simulink model "HFMA_4B_1_5_9_13"  (R2026b)
settings: Solver=FixedStepDiscrete  StopTime=stopTime  FixedStep=Ts
PreLoadFcn:
  | load('a_luts.mat')
values from neighbouring files (symbols this model uses):
  cosLUT = [1 1 1 1 1 1 1 1 1 1 1 1 ... (640 elements, 16x40)]    [iq_luts.mat]
  k_avg = 10    [Simulink_DOA_Test.m]    (also in collect_ranges.m; optimised_error_code.m)
  sinLUT = [0 0 0 0 0 0 0 0 0 0 0 0 ... (640 elements, 16x40)]    [iq_luts.mat]
  Ts = 1/8000    (= 0.000125)    [Simulink_DOA_Test.m]    (also in collect_ranges.m; optimised_error_code.m)
undefined symbols (not defined in the file or in its folder): a2_Im, a2_Re, a3_Im, a3_Re, NumBits1, NumBits2, Slope1, Slope2
libraries: hdlsllib x4, sl_signal_attributes x2
(part 1 of 6)
settings Model: FPTRunName=BaselineRun  FPTShortcutValueString='{{},{''BaselineRun_2'',1,1,1,''BaselineRun_2'','''',{},''M'',''D'',''''}}'  MinMaxOverflowArchiveMode=Merge  Creator=Kayla  LastModifiedBy=Kayla
settings OptimizationCC: BlockReduction=off  ConditionallyExecuteInputs=off  DefaultParameterBehavior=Inlined  InheritOutputTypeSmallerThanSingle=on
settings DebuggingCC: ArtificialAlgebraicLoopMsg=error  IntegerOverflowMsg=none  IntegerSaturationMsg=none  ParameterPrecisionLossMsg=none  SignalRangeChecking=warning  SingleTaskRateTransMsg=error
settings HardwareCC: ProdEndianess=Unspecified  ProdEqTarget=off  ProdHWDeviceType=ASIC/FPGA->ASIC/FPGA  ProdIntDivRoundTo=Undefined  ProdLargestAtomicFloat=None  TargetEndianess=LittleEndian  TargetHWDeviceType=Custom Processor->MATLAB Host Computer  TargetIntDivRoundTo=Zero  TargetLongLongMode=on

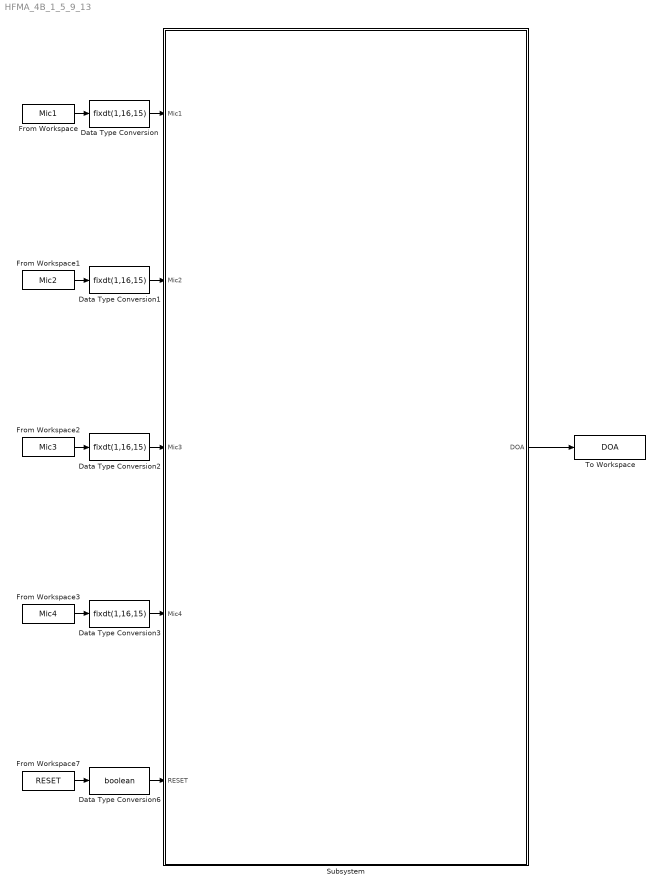
== system HFMA_4B_1_5_9_13 ==
  Data Type Conversion{,1..3} (4 alike) : DataTypeConversion  OutDataTypeStr=fixdt(1,16,15)  RndMeth=Nearest
  Data Type Conversion6 : DataTypeConversion  OutDataTypeStr=boolean  RndMeth=Nearest
  From Workspace : FromWorkspace  VariableName=Mic1  SampleTime=Ts  Interpolate=off  OutputAfterFinalValue=Holding final value
  From Workspace1 : FromWorkspace  VariableName=Mic2  SampleTime=Ts  Interpolate=off  OutputAfterFinalValue=Holding final value
  From Workspace2 : FromWorkspace  VariableName=Mic3  SampleTime=Ts  Interpolate=off  OutputAfterFinalValue=Holding final value
  From Workspace3 : FromWorkspace  VariableName=Mic4  SampleTime=Ts  Interpolate=off  OutputAfterFinalValue=Holding final value
  From Workspace7 : FromWorkspace  VariableName=RESET  SampleTime=Ts
  Subsystem : Subsystem
  To Workspace : ToWorkspace  VariableName=DOA  SaveFormat=Timeseries  SampleTime=-1
  wires:
  From Workspace7/1 -> Data Type Conversion6/1
  Subsystem/1(DOA) -> To Workspace/1
  From Workspace/1 -> Data Type Conversion/1
  From Workspace1/1 -> Data Type Conversion1/1
  From Workspace2/1 -> Data Type Conversion2/1
  From Workspace3/1 -> Data Type Conversion3/1
  Data Type Conversion/1 -> Subsystem/1(Mic1)
  Data Type Conversion1/1 -> Subsystem/2(Mic2)
  Data Type Conversion2/1 -> Subsystem/3(Mic3)
  Data Type Conversion3/1 -> Subsystem/4(Mic4)
  Data Type Conversion6/1 -> Subsystem/5(RESET)

== system HFMA_4B_1_5_9_13/Subsystem ==
  Mic1 : Inport  OutDataTypeStr=fixdt(1,16,15)  SampleTime=Ts
  Mic2 : Inport  Port=2  OutDataTypeStr=fixdt(1,16,15)  SampleTime=Ts
  Mic3 : Inport  Port=3  OutDataTypeStr=fixdt(1,16,15)  SampleTime=Ts
  Mic4 : Inport  Port=4  OutDataTypeStr=fixdt(1,16,15)  SampleTime=Ts
  RESET : Inport  Port=5  SampleTime=Ts
  A Counter : Subsystem  mask(Counter Limited){uplimit=180, tsamp=Ts}
      mask prompts: uplimit "Simulink:masks:UpperLimit_MP"; tsamp "Simulink:masks:SampleTime_MP"
      mask help: Simulink:masks:CounterLimited_MD
      mask init:
      | nbits = sl('counter_init', uplimit, gcbh);
  Add : Sum  Inputs=++++  OutDataTypeStr=fixdt(0,40,34)  SaturateOnIntegerOverflow=on
  Bandpass Filter : Subsystem
  Bandpass Filter1 : Subsystem
  Bandpass Filter2 : Subsystem
  Bandpass Filter3 : Subsystem
  Constant1 : Constant  OutDataTypeStr=fixdt(0,18,0)
  Constant13 : Constant  Value=13  OutDataTypeStr=fixdt(0,18,0)
  Constant5 : Constant  Value=5  OutDataTypeStr=fixdt(0,18,0)
  Constant9 : Constant  Value=9  OutDataTypeStr=fixdt(0,18,0)
  HFMA1 : Subsystem
  HFMA13 : Subsystem
  HFMA5 : Subsystem
  HFMA9 : Subsystem
  IQ Counter : Subsystem  mask(Counter Limited){uplimit=39, tsamp=Ts}
      mask prompts: uplimit "Simulink:masks:UpperLimit_MP"; tsamp "Simulink:masks:SampleTime_MP"
      mask help: Simulink:masks:CounterLimited_MD
      mask init:
      | nbits = sl('counter_init', uplimit, gcbh);
  Max Theta Selector : Subsystem
      settings: PortSchema="{\"entries\":[{\"content\":{\"sides\":[{\"content\":{\"connectorIds\":[\"In1\",\"In2\"]},\"type\":\"ConnectorPlacement.EquallySpacedRectSide\",\"uuid\":\"52f73d59-b961-46ba-95ec-da8ce9ae0879\"},{\"content\":{\"connectorIds\":[\"Out1\"],\"side\":\"RIGHT\"},\"type\":\"ConnectorPlacement.EquallySpacedRectSide\",\"uuid\":\"e217b0cb-9215-4a6d-97a8-b302314659a3\"},{\"content\":{\"connectorIds\":[\"In3\"],\"side\":\"TOP\"},\"type\":\"ConnectorPlacement.EquallySpacedRectSide\",\"uuid\":\"d49e545c-3ad9-445b-9897-a9fe5aaea0e6\"}]},\"type\":\"ConnectorPlacement.EquallySpacedConnector\",\"uuid\":\"e5954731-cd34-4517-a2ca-3982d6e46876\"}],\"packageUris\":[\"http://schema.mathworks.com/mf0/Connector/R2020b\"],\"version\":\"1.0\"}"
  DOA : Outport
  wires:
  Mic4/1 -> Bandpass Filter3/1(In1)
  Mic2/1 -> Bandpass Filter1/1(In1)
  Mic3/1 -> Bandpass Filter2/1(In1)
  Add/1 -> Max Theta Selector/1(P_Theta)
  Mic1/1 -> Bandpass Filter/1(Raw Signal In)
  Max Theta Selector/1(Strongest Angle) -> DOA/1
  Constant1/1 -> HFMA1/6(F0 Index)
  Constant5/1 -> HFMA5/6(F0 Index)
  Bandpass Filter/1(Filtered Output) -> HFMA1/1(Mic1), HFMA5/1(Mic1), HFMA9/1(Mic1), HFMA13/1(Mic1)
  Bandpass Filter1/1(Microphone Input) -> HFMA1/2(Mic2), HFMA5/2(Mic2), HFMA9/2(Mic2), HFMA13/2(Mic2)
  Bandpass Filter2/1(Microphone Input) -> HFMA1/3(Mic3), HFMA5/3(Mic3), HFMA9/3(Mic3), HFMA13/3(Mic3)
  Constant13/1 -> HFMA13/6(F0 Index)
  IQ Counter/1(y) -> HFMA1/7(IQ Counter), HFMA5/7(IQ Counter), HFMA9/7(IQ Counter), HFMA13/7(IQ Counter)
  A Counter/1(y) -> HFMA1/8(A Counter), HFMA5/8(A Counter), HFMA9/8(A Counter), HFMA13/8(A Counter)
  Constant9/1 -> HFMA9/6(F0 Index)
  Bandpass Filter3/1(Microphone Input) -> HFMA1/4(Mic4), HFMA5/4(Mic4), HFMA9/4(Mic4), HFMA13/4(Mic4)
  HFMA5/2(Theta) -> Max Theta Selector/2(Theta)
  RESET/1 -> Max Theta Selector/3(RESET), HFMA1/5(RESET), HFMA5/5(RESET), HFMA9/5(RESET), HFMA13/5(RESET)
  HFMA1/1(P_theta) -> Add/1
  HFMA5/1(P_theta) -> Add/2
  HFMA9/1(P_theta) -> Add/3
  HFMA13/1(P_theta) -> Add/4

== system HFMA_4B_1_5_9_13/Subsystem/A Counter ==
  Data Type Propagation : sl_signal_attributes/Data Type Propagation  PropDataTypeMode=Specify via dialog  PropDataType=uint(nbits)  IfRefDouble=double  IfRefSingle=single  IsSigned=IsSigned1 or IsSigned2  NumBitsBase=max([NumBits1 NumBits2])  NumBitsMult=1  NumBitsAdd=0  NumBitsAllowFinal=-1  PropScalingMode=Specify via dialog  PropScaling=1  ValuesUsedBestPrec=[5 -7]  SlopeBase=min([Slope1 Slope2])  SlopeMult=1  SlopeAdd=0  BiasBase=Bias1  BiasMult=1  BiasAdd=0
  Force to be scalar : SignalSpecification  DisableCoverage=on  Dimensions=1
  Increment Real World : hdlsllib/Math Operations/Increment Real World
  Output : UnitDelay  InitialCondition=0.0  SampleTime=tsamp
  Wrap To Zero : hdlsllib/Discontinuities/Wrap To Zero  Threshold=uplimit
  y : Outport
  wires:
  Increment Real World/1 -> Wrap To Zero/1
  Force to be scalar/1 -> Increment Real World/1
  Output/1 -> Force to be scalar/1, y/1
  Wrap To Zero/1 -> Output/1, Data Type Propagation/3, Data Type Propagation/2, Data Type Propagation/1

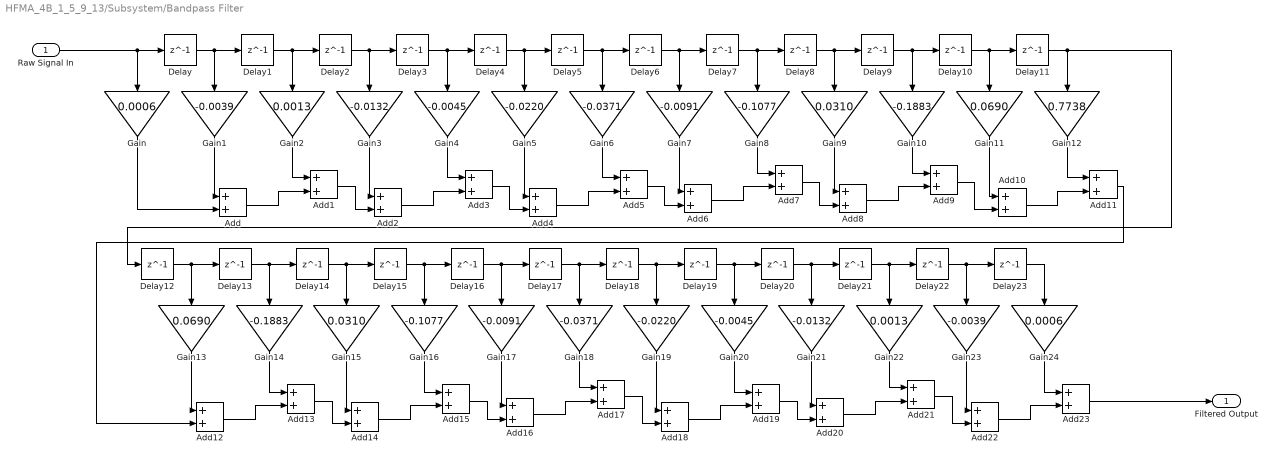
== system HFMA_4B_1_5_9_13/Subsystem/Bandpass Filter ==
  Raw Signal In : Inport
  Add{,1..23} (24 alike) : Sum  OutDataTypeStr=fixdt(1,20,17)  SaturateOnIntegerOverflow=on
  Delay{,1..23} (24 alike) : Delay  DelayLength=1
  Gain : Gain  Gain=0.0006  ParamDataTypeStr=fixdt(0,18,28)  OutDataTypeStr=fixdt(1,18,27)  SaturateOnIntegerOverflow=on
  Gain1 : Gain  Gain=-0.0039  ParamDataTypeStr=fixdt(1,18,25)  OutDataTypeStr=fixdt(1,18,24)  SaturateOnIntegerOverflow=on
  Gain10 : Gain  Gain=-0.1883  ParamDataTypeStr=fixdt(1,18,19)  OutDataTypeStr=fixdt(1,18,19)  SaturateOnIntegerOverflow=on
  Gain11 : Gain  Gain=0.0690  ParamDataTypeStr=fixdt(0,18,21)  OutDataTypeStr=fixdt(1,18,20)  SaturateOnIntegerOverflow=on
  Gain12 : Gain  Gain=0.7738  ParamDataTypeStr=fixdt(0,18,18)  OutDataTypeStr=fixdt(1,18,17)  SaturateOnIntegerOverflow=on
  Gain13 : Gain  Gain=0.0690  ParamDataTypeStr=fixdt(0,18,21)  OutDataTypeStr=fixdt(1,18,20)  SaturateOnIntegerOverflow=on
  Gain14 : Gain  Gain=-0.1883  ParamDataTypeStr=fixdt(1,18,19)  OutDataTypeStr=fixdt(1,18,19)  SaturateOnIntegerOverflow=on
  Gain15 : Gain  Gain=0.0310  ParamDataTypeStr=fixdt(0,18,23)  OutDataTypeStr=fixdt(1,18,21)  SaturateOnIntegerOverflow=on
  Gain16 : Gain  Gain=-0.1077  ParamDataTypeStr=fixdt(1,18,20)  OutDataTypeStr=fixdt(1,18,20)  SaturateOnIntegerOverflow=on
  Gain17 : Gain  Gain=-0.0091  ParamDataTypeStr=fixdt(1,18,23)  OutDataTypeStr=fixdt(1,18,23)  SaturateOnIntegerOverflow=on
  Gain18 : Gain  Gain=-0.0371  ParamDataTypeStr=fixdt(1,18,21)  OutDataTypeStr=fixdt(1,18,21)  SaturateOnIntegerOverflow=on
  Gain19 : Gain  Gain=-0.0220  ParamDataTypeStr=fixdt(1,18,22)  OutDataTypeStr=fixdt(1,18,22)  SaturateOnIntegerOverflow=on
  Gain2 : Gain  Gain=0.0013  ParamDataTypeStr=fixdt(0,18,27)  OutDataTypeStr=fixdt(1,18,26)  SaturateOnIntegerOverflow=on
  Gain20 : Gain  Gain=-0.0045  ParamDataTypeStr=fixdt(1,18,24)  OutDataTypeStr=fixdt(1,18,24)  SaturateOnIntegerOverflow=on
  Gain21 : Gain  Gain=-0.0132  ParamDataTypeStr=fixdt(1,18,23)  OutDataTypeStr=fixdt(1,18,23)  SaturateOnIntegerOverflow=on
  Gain22 : Gain  Gain=0.0013  ParamDataTypeStr=fixdt(0,18,27)  OutDataTypeStr=fixdt(1,18,26)  SaturateOnIntegerOverflow=on
  Gain23 : Gain  Gain=-0.0039  ParamDataTypeStr=fixdt(1,18,25)  OutDataTypeStr=fixdt(1,18,24)  SaturateOnIntegerOverflow=on
  Gain24 : Gain  Gain=0.0006  ParamDataTypeStr=fixdt(0,18,28)  OutDataTypeStr=fixdt(1,18,27)  SaturateOnIntegerOverflow=on
  Gain3 : Gain  Gain=-0.0132  ParamDataTypeStr=fixdt(1,18,23)  OutDataTypeStr=fixdt(1,18,23)  SaturateOnIntegerOverflow=on
  Gain4 : Gain  Gain=-0.0045  ParamDataTypeStr=fixdt(1,18,24)  OutDataTypeStr=fixdt(1,18,24)  SaturateOnIntegerOverflow=on
  Gain5 : Gain  Gain=-0.0220  ParamDataTypeStr=fixdt(1,18,22)  OutDataTypeStr=fixdt(1,18,22)  SaturateOnIntegerOverflow=on
  Gain6 : Gain  Gain=-0.0371  ParamDataTypeStr=fixdt(1,18,21)  OutDataTypeStr=fixdt(1,18,21)  SaturateOnIntegerOverflow=on
  Gain7 : Gain  Gain=-0.0091  ParamDataTypeStr=fixdt(1,18,23)  OutDataTypeStr=fixdt(1,18,23)  SaturateOnIntegerOverflow=on
  Gain8 : Gain  Gain=-0.1077  ParamDataTypeStr=fixdt(1,18,20)  OutDataTypeStr=fixdt(1,18,20)  SaturateOnIntegerOverflow=on
  Gain9 : Gain  Gain=0.0310  ParamDataTypeStr=fixdt(0,18,23)  OutDataTypeStr=fixdt(1,18,21)  SaturateOnIntegerOverflow=on
  Filtered Output : Outport
  wires:
  Gain6/1 -> Add5/1
  Delay13/1 -> Delay14/1, Gain14/1
  Delay20/1 -> Delay21/1, Gain21/1
  Delay11/1 -> Gain12/1, Delay12/1
  Raw Signal In/1 -> Delay/1, Gain/1
  Add9/1 -> Add10/2
  Delay/1 -> Delay1/1, Gain1/1
  Delay1/1 -> Delay2/1, Gain2/1
  Add14/1 -> Add15/2
  Gain22/1 -> Add21/1
  Delay3/1 -> Delay4/1, Gain4/1
  Delay14/1 -> Delay15/1, Gain15/1
  Delay19/1 -> Delay20/1, Gain20/1
  Delay5/1 -> Delay6/1, Gain6/1
  Delay2/1 -> Delay3/1, Gain3/1
  Delay21/1 -> Delay22/1, Gain22/1
  Delay6/1 -> Delay7/1, Gain7/1
  Delay4/1 -> Delay5/1, Gain5/1
  Delay18/1 -> Delay19/1, Gain19/1
  Gain14/1 -> Add13/1
  Delay10/1 -> Delay11/1, Gain11/1
  Delay12/1 -> Delay13/1, Gain13/1
  Gain2/1 -> Add1/1
  Delay15/1 -> Delay16/1, Gain16/1
  Delay7/1 -> Delay8/1, Gain8/1
  Delay8/1 -> Delay9/1, Gain9/1
  Add20/1 -> Add21/2
  Delay9/1 -> Delay10/1, Gain10/1
  Add7/1 -> Add8/2
  Add1/1 -> Add2/2
  Delay16/1 -> Delay17/1, Gain17/1
  Add8/1 -> Add9/2
  Delay17/1 -> Delay18/1, Gain18/1
  Gain21/1 -> Add20/1
  Add5/1 -> Add6/2
  Delay23/1 -> Gain24/1
  Add17/1 -> Add18/2
  Gain15/1 -> Add14/1
  Gain4/1 -> Add3/1
  Gain3/1 -> Add2/1
  Delay22/1 -> Delay23/1, Gain23/1
  Gain/1 -> Add/2
  Add13/1 -> Add14/2
  Add15/1 -> Add16/2
  Gain1/1 -> Add/1
  Gain24/1 -> Add23/1
  Gain5/1 -> Add4/1
  Gain11/1 -> Add10/1
  Gain7/1 -> Add6/1
  Gain19/1 -> Add18/1
  Gain8/1 -> Add7/1
  Gain9/1 -> Add8/1
  Add11/1 -> Add12/2
  Gain10/1 -> Add9/1
  Add21/1 -> Add22/2
  Gain12/1 -> Add11/1
  Gain13/1 -> Add12/1
  Gain16/1 -> Add15/1
  Gain17/1 -> Add16/1
  Gain18/1 -> Add17/1
  Gain20/1 -> Add19/1
  Gain23/1 -> Add22/1
  Add3/1 -> Add4/2
  Add19/1 -> Add20/2
  Add23/1 -> Filtered Output/1
  Add6/1 -> Add7/2
  Add16/1 -> Add17/2
  Add/1 -> Add1/2
  Add2/1 -> Add3/2
  Add4/1 -> Add5/2
  Add10/1 -> Add11/2
  Add12/1 -> Add13/2
  Add18/1 -> Add19/2
  Add22/1 -> Add23/2

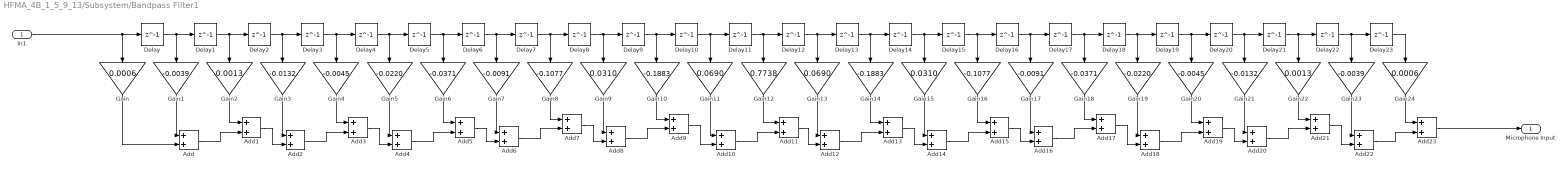
== system HFMA_4B_1_5_9_13/Subsystem/Bandpass Filter1 ==
  In1 : Inport
  Add{,1..23} (24 alike) : Sum  OutDataTypeStr=fixdt(1,20,17)  SaturateOnIntegerOverflow=on
  Delay{,1..23} (24 alike) : Delay  DelayLength=1
  Gain : Gain  Gain=0.0006  ParamDataTypeStr=fixdt(0,18,28)  OutDataTypeStr=fixdt(1,18,27)  SaturateOnIntegerOverflow=on
  Gain1 : Gain  Gain=-0.0039  ParamDataTypeStr=fixdt(1,18,25)  OutDataTypeStr=fixdt(1,18,24)  SaturateOnIntegerOverflow=on
  Gain10 : Gain  Gain=-0.1883  ParamDataTypeStr=fixdt(1,18,19)  OutDataTypeStr=fixdt(1,18,19)  SaturateOnIntegerOverflow=on
  Gain11 : Gain  Gain=0.0690  ParamDataTypeStr=fixdt(0,18,21)  OutDataTypeStr=fixdt(1,18,20)  SaturateOnIntegerOverflow=on
  Gain12 : Gain  Gain=0.7738  ParamDataTypeStr=fixdt(0,18,18)  OutDataTypeStr=fixdt(1,18,17)  SaturateOnIntegerOverflow=on
  Gain13 : Gain  Gain=0.0690  ParamDataTypeStr=fixdt(0,18,21)  OutDataTypeStr=fixdt(1,18,20)  SaturateOnIntegerOverflow=on
  Gain14 : Gain  Gain=-0.1883  ParamDataTypeStr=fixdt(1,18,19)  OutDataTypeStr=fixdt(1,18,19)  SaturateOnIntegerOverflow=on
  Gain15 : Gain  Gain=0.0310  ParamDataTypeStr=fixdt(0,18,23)  OutDataTypeStr=fixdt(1,18,21)  SaturateOnIntegerOverflow=on
  Gain16 : Gain  Gain=-0.1077  ParamDataTypeStr=fixdt(1,18,20)  OutDataTypeStr=fixdt(1,18,20)  SaturateOnIntegerOverflow=on
  Gain17 : Gain  Gain=-0.0091  ParamDataTypeStr=fixdt(1,18,23)  OutDataTypeStr=fixdt(1,18,23)  SaturateOnIntegerOverflow=on
  Gain18 : Gain  Gain=-0.0371  ParamDataTypeStr=fixdt(1,18,21)  OutDataTypeStr=fixdt(1,18,21)  SaturateOnIntegerOverflow=on
  Gain19 : Gain  Gain=-0.0220  ParamDataTypeStr=fixdt(1,18,22)  OutDataTypeStr=fixdt(1,18,22)  SaturateOnIntegerOverflow=on
  Gain2 : Gain  Gain=0.0013  ParamDataTypeStr=fixdt(0,18,27)  OutDataTypeStr=fixdt(1,18,26)  SaturateOnIntegerOverflow=on
  Gain20 : Gain  Gain=-0.0045  ParamDataTypeStr=fixdt(1,18,24)  OutDataTypeStr=fixdt(1,18,24)  SaturateOnIntegerOverflow=on
  Gain21 : Gain  Gain=-0.0132  ParamDataTypeStr=fixdt(1,18,23)  OutDataTypeStr=fixdt(1,18,23)  SaturateOnIntegerOverflow=on
  Gain22 : Gain  Gain=0.0013  ParamDataTypeStr=fixdt(0,18,27)  OutDataTypeStr=fixdt(1,18,26)  SaturateOnIntegerOverflow=on
  Gain23 : Gain  Gain=-0.0039  ParamDataTypeStr=fixdt(1,18,25)  OutDataTypeStr=fixdt(1,18,24)  SaturateOnIntegerOverflow=on
  Gain24 : Gain  Gain=0.0006  ParamDataTypeStr=fixdt(0,18,28)  OutDataTypeStr=fixdt(1,18,27)  SaturateOnIntegerOverflow=on
  Gain3 : Gain  Gain=-0.0132  ParamDataTypeStr=fixdt(1,18,23)  OutDataTypeStr=fixdt(1,18,23)  SaturateOnIntegerOverflow=on
  Gain4 : Gain  Gain=-0.0045  ParamDataTypeStr=fixdt(1,18,24)  OutDataTypeStr=fixdt(1,18,24)  SaturateOnIntegerOverflow=on
  Gain5 : Gain  Gain=-0.0220  ParamDataTypeStr=fixdt(1,18,22)  OutDataTypeStr=fixdt(1,18,22)  SaturateOnIntegerOverflow=on
  Gain6 : Gain  Gain=-0.0371  ParamDataTypeStr=fixdt(1,18,21)  OutDataTypeStr=fixdt(1,18,21)  SaturateOnIntegerOverflow=on
  Gain7 : Gain  Gain=-0.0091  ParamDataTypeStr=fixdt(1,18,23)  OutDataTypeStr=fixdt(1,18,23)  SaturateOnIntegerOverflow=on
  Gain8 : Gain  Gain=-0.1077  ParamDataTypeStr=fixdt(1,18,20)  OutDataTypeStr=fixdt(1,18,20)  SaturateOnIntegerOverflow=on
  Gain9 : Gain  Gain=0.0310  ParamDataTypeStr=fixdt(0,18,23)  OutDataTypeStr=fixdt(1,18,21)  SaturateOnIntegerOverflow=on
  Microphone Input : Outport
  wires:
  Gain6/1 -> Add5/1
  Delay13/1 -> Delay14/1, Gain14/1
  Delay20/1 -> Delay21/1, Gain21/1
  Delay11/1 -> Delay12/1, Gain12/1
  In1/1 -> Delay/1, Gain/1
  Add9/1 -> Add10/2
  Delay/1 -> Delay1/1, Gain1/1
  Delay1/1 -> Delay2/1, Gain2/1
  Add14/1 -> Add15/2
  Gain22/1 -> Add21/1
  Delay3/1 -> Delay4/1, Gain4/1
  Delay14/1 -> Delay15/1, Gain15/1
  Delay19/1 -> Delay20/1, Gain20/1
  Delay5/1 -> Delay6/1, Gain6/1
  Delay2/1 -> Delay3/1, Gain3/1
  Delay21/1 -> Delay22/1, Gain22/1
  Delay6/1 -> Delay7/1, Gain7/1
  Delay4/1 -> Delay5/1, Gain5/1
  Delay18/1 -> Delay19/1, Gain19/1
  Gain14/1 -> Add13/1
  Delay10/1 -> Delay11/1, Gain11/1
  Delay12/1 -> Delay13/1, Gain13/1
  Gain2/1 -> Add1/1
  Delay15/1 -> Delay16/1, Gain16/1
  Delay7/1 -> Delay8/1, Gain8/1
  Delay8/1 -> Delay9/1, Gain9/1
  Add20/1 -> Add21/2
  Delay9/1 -> Delay10/1, Gain10/1
  Add7/1 -> Add8/2
  Add1/1 -> Add2/2
  Delay16/1 -> Delay17/1, Gain17/1
  Add8/1 -> Add9/2
  Delay17/1 -> Delay18/1, Gain18/1
  Gain21/1 -> Add20/1
  Add5/1 -> Add6/2
  Delay23/1 -> Gain24/1
  Add17/1 -> Add18/2
  Gain15/1 -> Add14/1
  Gain4/1 -> Add3/1
  Gain3/1 -> Add2/1
  Delay22/1 -> Delay23/1, Gain23/1
  Gain/1 -> Add/2
  Add13/1 -> Add14/2
  Add15/1 -> Add16/2
  Gain1/1 -> Add/1
  Gain24/1 -> Add23/1
  Gain5/1 -> Add4/1
  Gain11/1 -> Add10/1
  Gain7/1 -> Add6/1
  Gain19/1 -> Add18/1
  Gain8/1 -> Add7/1
  Gain9/1 -> Add8/1
  Add11/1 -> Add12/2
  Gain10/1 -> Add9/1
  Add21/1 -> Add22/2
  Gain12/1 -> Add11/1
  Gain13/1 -> Add12/1
  Gain16/1 -> Add15/1
  Gain17/1 -> Add16/1
  Gain18/1 -> Add17/1
  Gain20/1 -> Add19/1
  Gain23/1 -> Add22/1
  Add3/1 -> Add4/2
  Add19/1 -> Add20/2
  Add23/1 -> Microphone Input/1
  Add6/1 -> Add7/2
  Add16/1 -> Add17/2
  Add/1 -> Add1/2
  Add2/1 -> Add3/2
  Add4/1 -> Add5/2
  Add10/1 -> Add11/2
  Add12/1 -> Add13/2
  Add18/1 -> Add19/2
  Add22/1 -> Add23/2

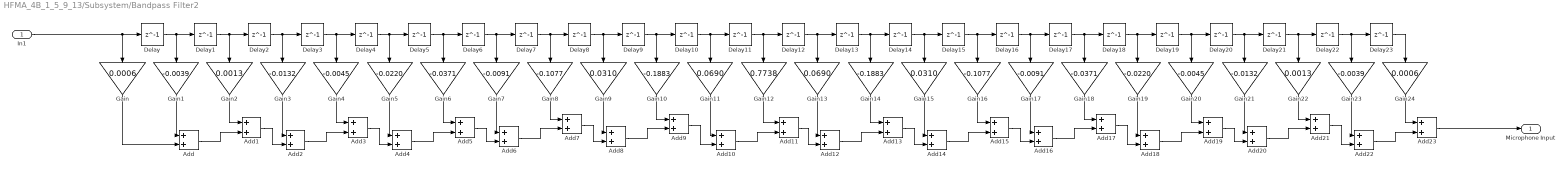
== system HFMA_4B_1_5_9_13/Subsystem/Bandpass Filter2 ==
  In1 : Inport
  Add{,1..23} (24 alike) : Sum  OutDataTypeStr=fixdt(1,20,17)  SaturateOnIntegerOverflow=on
  Delay{,1..23} (24 alike) : Delay  DelayLength=1
  Gain : Gain  Gain=0.0006  ParamDataTypeStr=fixdt(0,18,28)  OutDataTypeStr=fixdt(1,18,27)  SaturateOnIntegerOverflow=on
  Gain1 : Gain  Gain=-0.0039  ParamDataTypeStr=fixdt(1,18,25)  OutDataTypeStr=fixdt(1,18,24)  SaturateOnIntegerOverflow=on
  Gain10 : Gain  Gain=-0.1883  ParamDataTypeStr=fixdt(1,18,19)  OutDataTypeStr=fixdt(1,18,19)  SaturateOnIntegerOverflow=on
  Gain11 : Gain  Gain=0.0690  ParamDataTypeStr=fixdt(0,18,21)  OutDataTypeStr=fixdt(1,18,20)  SaturateOnIntegerOverflow=on
  Gain12 : Gain  Gain=0.7738  ParamDataTypeStr=fixdt(0,18,18)  OutDataTypeStr=fixdt(1,18,17)  SaturateOnIntegerOverflow=on
  Gain13 : Gain  Gain=0.0690  ParamDataTypeStr=fixdt(0,18,21)  OutDataTypeStr=fixdt(1,18,20)  SaturateOnIntegerOverflow=on
  Gain14 : Gain  Gain=-0.1883  ParamDataTypeStr=fixdt(1,18,19)  OutDataTypeStr=fixdt(1,18,19)  SaturateOnIntegerOverflow=on
  Gain15 : Gain  Gain=0.0310  ParamDataTypeStr=fixdt(0,18,23)  OutDataTypeStr=fixdt(1,18,21)  SaturateOnIntegerOverflow=on
  Gain16 : Gain  Gain=-0.1077  ParamDataTypeStr=fixdt(1,18,20)  OutDataTypeStr=fixdt(1,18,20)  SaturateOnIntegerOverflow=on
  Gain17 : Gain  Gain=-0.0091  ParamDataTypeStr=fixdt(1,18,23)  OutDataTypeStr=fixdt(1,18,23)  SaturateOnIntegerOverflow=on
  Gain18 : Gain  Gain=-0.0371  ParamDataTypeStr=fixdt(1,18,21)  OutDataTypeStr=fixdt(1,18,21)  SaturateOnIntegerOverflow=on
  Gain19 : Gain  Gain=-0.0220  ParamDataTypeStr=fixdt(1,18,22)  OutDataTypeStr=fixdt(1,18,22)  SaturateOnIntegerOverflow=on
  Gain2 : Gain  Gain=0.0013  ParamDataTypeStr=fixdt(0,18,27)  OutDataTypeStr=fixdt(1,18,26)  SaturateOnIntegerOverflow=on
  Gain20 : Gain  Gain=-0.0045  ParamDataTypeStr=fixdt(1,18,24)  OutDataTypeStr=fixdt(1,18,24)  SaturateOnIntegerOverflow=on
  Gain21 : Gain  Gain=-0.0132  ParamDataTypeStr=fixdt(1,18,23)  OutDataTypeStr=fixdt(1,18,23)  SaturateOnIntegerOverflow=on
  Gain22 : Gain  Gain=0.0013  ParamDataTypeStr=fixdt(0,18,27)  OutDataTypeStr=fixdt(1,18,26)  SaturateOnIntegerOverflow=on
  Gain23 : Gain  Gain=-0.0039  ParamDataTypeStr=fixdt(1,18,25)  OutDataTypeStr=fixdt(1,18,24)  SaturateOnIntegerOverflow=on
  Gain24 : Gain  Gain=0.0006  ParamDataTypeStr=fixdt(0,18,28)  OutDataTypeStr=fixdt(1,18,27)  SaturateOnIntegerOverflow=on
  Gain3 : Gain  Gain=-0.0132  ParamDataTypeStr=fixdt(1,18,23)  OutDataTypeStr=fixdt(1,18,23)  SaturateOnIntegerOverflow=on
  Gain4 : Gain  Gain=-0.0045  ParamDataTypeStr=fixdt(1,18,24)  OutDataTypeStr=fixdt(1,18,24)  SaturateOnIntegerOverflow=on
  Gain5 : Gain  Gain=-0.0220  ParamDataTypeStr=fixdt(1,18,22)  OutDataTypeStr=fixdt(1,18,22)  SaturateOnIntegerOverflow=on
  Gain6 : Gain  Gain=-0.0371  ParamDataTypeStr=fixdt(1,18,21)  OutDataTypeStr=fixdt(1,18,21)  SaturateOnIntegerOverflow=on
  Gain7 : Gain  Gain=-0.0091  ParamDataTypeStr=fixdt(1,18,23)  OutDataTypeStr=fixdt(1,18,23)  SaturateOnIntegerOverflow=on
  Gain8 : Gain  Gain=-0.1077  ParamDataTypeStr=fixdt(1,18,20)  OutDataTypeStr=fixdt(1,18,20)  SaturateOnIntegerOverflow=on
  Gain9 : Gain  Gain=0.0310  ParamDataTypeStr=fixdt(0,18,23)  OutDataTypeStr=fixdt(1,18,21)  SaturateOnIntegerOverflow=on
  Microphone Input : Outport
  wires:
  Gain6/1 -> Add5/1
  Delay13/1 -> Delay14/1, Gain14/1
  Delay20/1 -> Delay21/1, Gain21/1
  Delay11/1 -> Delay12/1, Gain12/1
  In1/1 -> Delay/1, Gain/1
  Add9/1 -> Add10/2
  Delay/1 -> Delay1/1, Gain1/1
  Delay1/1 -> Delay2/1, Gain2/1
  Add14/1 -> Add15/2
  Gain22/1 -> Add21/1
  Delay3/1 -> Delay4/1, Gain4/1
  Delay14/1 -> Delay15/1, Gain15/1
  Delay19/1 -> Delay20/1, Gain20/1
  Delay5/1 -> Delay6/1, Gain6/1
  Delay2/1 -> Delay3/1, Gain3/1
  Delay21/1 -> Delay22/1, Gain22/1
  Delay6/1 -> Delay7/1, Gain7/1
  Delay4/1 -> Delay5/1, Gain5/1
  Delay18/1 -> Delay19/1, Gain19/1
  Gain14/1 -> Add13/1
  Delay10/1 -> Delay11/1, Gain11/1
  Delay12/1 -> Delay13/1, Gain13/1
  Gain2/1 -> Add1/1
  Delay15/1 -> Delay16/1, Gain16/1
  Delay7/1 -> Delay8/1, Gain8/1
  Delay8/1 -> Delay9/1, Gain9/1
  Add20/1 -> Add21/2
  Delay9/1 -> Delay10/1, Gain10/1
  Add7/1 -> Add8/2
  Add1/1 -> Add2/2
  Delay16/1 -> Delay17/1, Gain17/1
  Add8/1 -> Add9/2
  Delay17/1 -> Delay18/1, Gain18/1
  Gain21/1 -> Add20/1
  Add5/1 -> Add6/2
  Delay23/1 -> Gain24/1
  Add17/1 -> Add18/2
  Gain15/1 -> Add14/1
  Gain4/1 -> Add3/1
  Gain3/1 -> Add2/1
  Delay22/1 -> Delay23/1, Gain23/1
  Gain/1 -> Add/2
  Add13/1 -> Add14/2
  Add15/1 -> Add16/2
  Gain1/1 -> Add/1
  Gain24/1 -> Add23/1
  Gain5/1 -> Add4/1
  Gain11/1 -> Add10/1
  Gain7/1 -> Add6/1
  Gain19/1 -> Add18/1
  Gain8/1 -> Add7/1
  Gain9/1 -> Add8/1
  Add11/1 -> Add12/2
  Gain10/1 -> Add9/1
  Add21/1 -> Add22/2
  Gain12/1 -> Add11/1
  Gain13/1 -> Add12/1
  Gain16/1 -> Add15/1
  Gain17/1 -> Add16/1
  Gain18/1 -> Add17/1
  Gain20/1 -> Add19/1
  Gain23/1 -> Add22/1
  Add3/1 -> Add4/2
  Add19/1 -> Add20/2
  Add23/1 -> Microphone Input/1
  Add6/1 -> Add7/2
  Add16/1 -> Add17/2
  Add/1 -> Add1/2
  Add2/1 -> Add3/2
  Add4/1 -> Add5/2
  Add10/1 -> Add11/2
  Add12/1 -> Add13/2
  Add18/1 -> Add19/2
  Add22/1 -> Add23/2

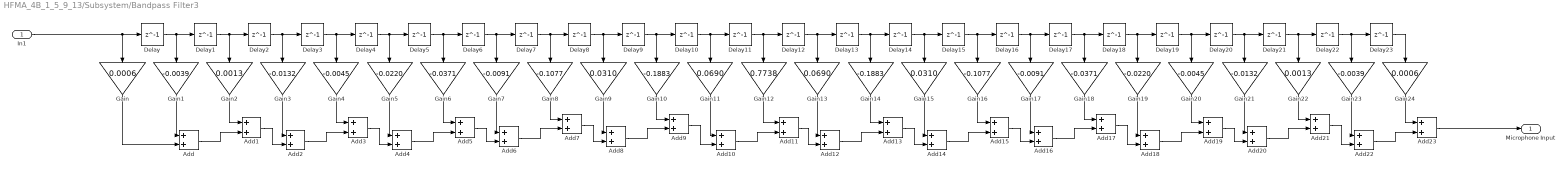
== system HFMA_4B_1_5_9_13/Subsystem/Bandpass Filter3 ==
  In1 : Inport
  Add{,1..23} (24 alike) : Sum  OutDataTypeStr=fixdt(1,20,17)  SaturateOnIntegerOverflow=on
  Delay{,1..23} (24 alike) : Delay  DelayLength=1
  Gain : Gain  Gain=0.0006  ParamDataTypeStr=fixdt(0,18,28)  OutDataTypeStr=fixdt(1,18,27)  SaturateOnIntegerOverflow=on
  Gain1 : Gain  Gain=-0.0039  ParamDataTypeStr=fixdt(1,18,25)  OutDataTypeStr=fixdt(1,18,24)  SaturateOnIntegerOverflow=on
  Gain10 : Gain  Gain=-0.1883  ParamDataTypeStr=fixdt(1,18,19)  OutDataTypeStr=fixdt(1,18,19)  SaturateOnIntegerOverflow=on
  Gain11 : Gain  Gain=0.0690  ParamDataTypeStr=fixdt(0,18,21)  OutDataTypeStr=fixdt(1,18,20)  SaturateOnIntegerOverflow=on
  Gain12 : Gain  Gain=0.7738  ParamDataTypeStr=fixdt(0,18,18)  OutDataTypeStr=fixdt(1,18,17)  SaturateOnIntegerOverflow=on
  Gain13 : Gain  Gain=0.0690  ParamDataTypeStr=fixdt(0,18,21)  OutDataTypeStr=fixdt(1,18,20)  SaturateOnIntegerOverflow=on
  Gain14 : Gain  Gain=-0.1883  ParamDataTypeStr=fixdt(1,18,19)  OutDataTypeStr=fixdt(1,18,19)  SaturateOnIntegerOverflow=on
  Gain15 : Gain  Gain=0.0310  ParamDataTypeStr=fixdt(0,18,23)  OutDataTypeStr=fixdt(1,18,21)  SaturateOnIntegerOverflow=on
  Gain16 : Gain  Gain=-0.1077  ParamDataTypeStr=fixdt(1,18,20)  OutDataTypeStr=fixdt(1,18,20)  SaturateOnIntegerOverflow=on
  Gain17 : Gain  Gain=-0.0091  ParamDataTypeStr=fixdt(1,18,23)  OutDataTypeStr=fixdt(1,18,23)  SaturateOnIntegerOverflow=on
  Gain18 : Gain  Gain=-0.0371  ParamDataTypeStr=fixdt(1,18,21)  OutDataTypeStr=fixdt(1,18,21)  SaturateOnIntegerOverflow=on
  Gain19 : Gain  Gain=-0.0220  ParamDataTypeStr=fixdt(1,18,22)  OutDataTypeStr=fixdt(1,18,22)  SaturateOnIntegerOverflow=on
  Gain2 : Gain  Gain=0.0013  ParamDataTypeStr=fixdt(0,18,27)  OutDataTypeStr=fixdt(1,18,26)  SaturateOnIntegerOverflow=on
  Gain20 : Gain  Gain=-0.0045  ParamDataTypeStr=fixdt(1,18,24)  OutDataTypeStr=fixdt(1,18,24)  SaturateOnIntegerOverflow=on
  Gain21 : Gain  Gain=-0.0132  ParamDataTypeStr=fixdt(1,18,23)  OutDataTypeStr=fixdt(1,18,23)  SaturateOnIntegerOverflow=on
  Gain22 : Gain  Gain=0.0013  ParamDataTypeStr=fixdt(0,18,27)  OutDataTypeStr=fixdt(1,18,26)  SaturateOnIntegerOverflow=on
  Gain23 : Gain  Gain=-0.0039  ParamDataTypeStr=fixdt(1,18,25)  OutDataTypeStr=fixdt(1,18,24)  SaturateOnIntegerOverflow=on
  Gain24 : Gain  Gain=0.0006  ParamDataTypeStr=fixdt(0,18,28)  OutDataTypeStr=fixdt(1,18,27)  SaturateOnIntegerOverflow=on
  Gain3 : Gain  Gain=-0.0132  ParamDataTypeStr=fixdt(1,18,23)  OutDataTypeStr=fixdt(1,18,23)  SaturateOnIntegerOverflow=on
  Gain4 : Gain  Gain=-0.0045  ParamDataTypeStr=fixdt(1,18,24)  OutDataTypeStr=fixdt(1,18,24)  SaturateOnIntegerOverflow=on
  Gain5 : Gain  Gain=-0.0220  ParamDataTypeStr=fixdt(1,18,22)  OutDataTypeStr=fixdt(1,18,22)  SaturateOnIntegerOverflow=on
  Gain6 : Gain  Gain=-0.0371  ParamDataTypeStr=fixdt(1,18,21)  OutDataTypeStr=fixdt(1,18,21)  SaturateOnIntegerOverflow=on
  Gain7 : Gain  Gain=-0.0091  ParamDataTypeStr=fixdt(1,18,23)  OutDataTypeStr=fixdt(1,18,23)  SaturateOnIntegerOverflow=on
  Gain8 : Gain  Gain=-0.1077  ParamDataTypeStr=fixdt(1,18,20)  OutDataTypeStr=fixdt(1,18,20)  SaturateOnIntegerOverflow=on
  Gain9 : Gain  Gain=0.0310  ParamDataTypeStr=fixdt(0,18,23)  OutDataTypeStr=fixdt(1,18,21)  SaturateOnIntegerOverflow=on
  Microphone Input : Outport
  wires:
  Gain6/1 -> Add5/1
  Delay13/1 -> Delay14/1, Gain14/1
  Delay20/1 -> Delay21/1, Gain21/1
  Delay11/1 -> Delay12/1, Gain12/1
  In1/1 -> Delay/1, Gain/1
  Add9/1 -> Add10/2
  Delay/1 -> Delay1/1, Gain1/1
  Delay1/1 -> Delay2/1, Gain2/1
  Add14/1 -> Add15/2
  Gain22/1 -> Add21/1
  Delay3/1 -> Delay4/1, Gain4/1
  Delay14/1 -> Delay15/1, Gain15/1
  Delay19/1 -> Delay20/1, Gain20/1
  Delay5/1 -> Delay6/1, Gain6/1
  Delay2/1 -> Delay3/1, Gain3/1
  Delay21/1 -> Delay22/1, Gain22/1
  Delay6/1 -> Delay7/1, Gain7/1
  Delay4/1 -> Delay5/1, Gain5/1
  Delay18/1 -> Delay19/1, Gain19/1
  Gain14/1 -> Add13/1
  Delay10/1 -> Delay11/1, Gain11/1
  Delay12/1 -> Delay13/1, Gain13/1
  Gain2/1 -> Add1/1
  Delay15/1 -> Delay16/1, Gain16/1
  Delay7/1 -> Delay8/1, Gain8/1
  Delay8/1 -> Delay9/1, Gain9/1
  Add20/1 -> Add21/2
  Delay9/1 -> Delay10/1, Gain10/1
  Add7/1 -> Add8/2
  Add1/1 -> Add2/2
  Delay16/1 -> Delay17/1, Gain17/1
  Add8/1 -> Add9/2
  Delay17/1 -> Delay18/1, Gain18/1
  Gain21/1 -> Add20/1
  Add5/1 -> Add6/2
  Delay23/1 -> Gain24/1
  Add17/1 -> Add18/2
  Gain15/1 -> Add14/1
  Gain4/1 -> Add3/1
  Gain3/1 -> Add2/1
  Delay22/1 -> Delay23/1, Gain23/1
  Gain/1 -> Add/2
  Add13/1 -> Add14/2
  Add15/1 -> Add16/2
  Gain1/1 -> Add/1
  Gain24/1 -> Add23/1
  Gain5/1 -> Add4/1
  Gain11/1 -> Add10/1
  Gain7/1 -> Add6/1
  Gain19/1 -> Add18/1
  Gain8/1 -> Add7/1
  Gain9/1 -> Add8/1
  Add11/1 -> Add12/2
  Gain10/1 -> Add9/1
  Add21/1 -> Add22/2
  Gain12/1 -> Add11/1
  Gain13/1 -> Add12/1
  Gain16/1 -> Add15/1
  Gain17/1 -> Add16/1
  Gain18/1 -> Add17/1
  Gain20/1 -> Add19/1
  Gain23/1 -> Add22/1
  Add3/1 -> Add4/2
  Add19/1 -> Add20/2
  Add23/1 -> Microphone Input/1
  Add6/1 -> Add7/2
  Add16/1 -> Add17/2
  Add/1 -> Add1/2
  Add2/1 -> Add3/2
  Add4/1 -> Add5/2
  Add10/1 -> Add11/2
  Add12/1 -> Add13/2
  Add18/1 -> Add19/2
  Add22/1 -> Add23/2

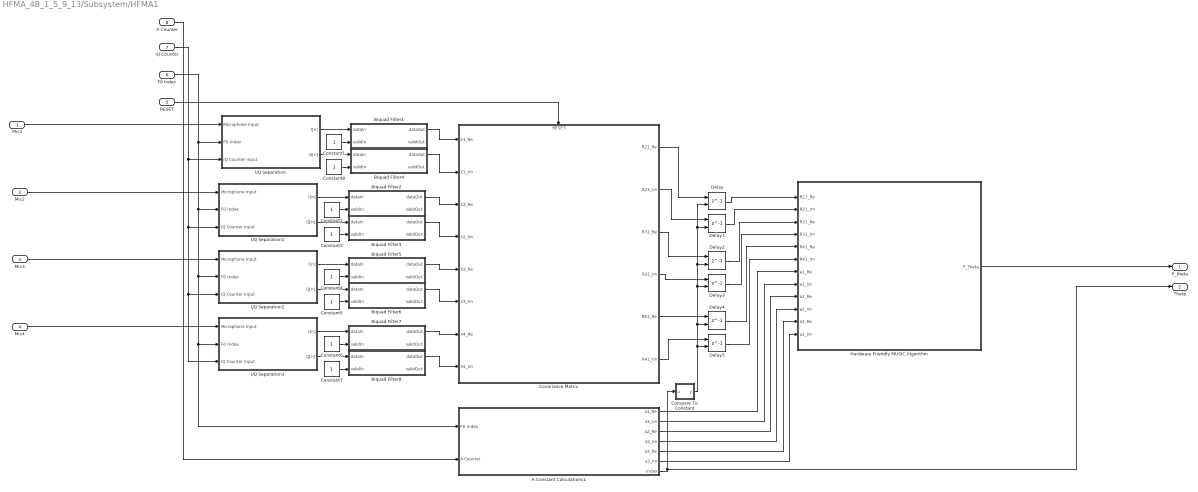
== system HFMA_4B_1_5_9_13/Subsystem/HFMA1 ==
  Mic1 : Inport
  Mic2 : Inport  Port=2
  Mic3 : Inport  Port=3
  Mic4 : Inport  Port=4
  RESET : Inport  Port=5
  F0 Index : Inport  Port=6
  IQ Counter : Inport  Port=7
  A Counter : Inport  Port=8
  A Constant Calculations1 : Subsystem
  Biquad Filter1 : Subsystem
  Biquad Filter2 : Subsystem
  Biquad Filter3 : Subsystem
  Biquad Filter4 : Subsystem
  Biquad Filter5 : Subsystem
  Biquad Filter6 : Subsystem
  Biquad Filter7 : Subsystem
  Biquad Filter8 : Subsystem
  Compare To Constant : Subsystem  mask(Compare To Constant){relop===, const=180, OutDataTypeStr=boolean, ZeroCross=on}
      mask prompts: relop "Simulink:masks:Operator_MP"; const "Simulink:masks:ConstantValue_MP"; OutDataTypeStr "Simulink:masks:OutputDataType_MP"; ZeroCross "Simulink:masks:EnableZerocrossingDetection_MP"
      mask help: Simulink:masks:CompareToConstant_MD
      mask init:
      | blkName = gcb;
      | 
      | if strcmp(get_param(gcbh,'OutDataTypeStr'),'boolean')
      | 	setValue = 'boolean';
      | else
      | 	setValue = 'fixdt(0, 8)';
      | end
      | 
      | set_param([blkName,'/Compare'],'relop',relop, ...
      | 	'OutDataTypeStr', setValue, 'ZeroCross', ZeroCross);
      | 
      | str = [relop,' C']; %default
      | 
      | const_str = get_param(blkName, 'const');
      | const_val = str2num(const_str);
      | 
      | if isempty(const_val) %#ok<ST2NM>
      |     %Expression/Variable
      |     str = [relop, ' ', strtrim(const_str)];
      | else
      |     if length(const_val) == 1 
      |         if Simulink.data.isSupportedEnumClass(class(const_val))
      |             % Special Handling for Enumerations
      |             if Simulink.data.getEnumTypeInfo(class(const_val), 'AddClassNameToEnumNames')
      |                 str = [relop, ' ', strtrim(const_str)];
      |             else
      |                 str = [relop, ' ', char(const_val)];
      |             end
      |         elseif(isfloat(const_val) || isinteger(const_val) || islogical(const_val)) 
      |                 str = [relop, ' ', num2str(const_val)];
      |         end
      |     end
      | end
      mask TypeOptions relop: == | ~= | < | <= | >= | >
      mask TypeOptions OutDataTypeStr: Simulink:masks:uint8 | Simulink:masks:boolean
      mask Callback ZeroCross: sl('zeroCrossEnable', gcbh);
      mask DialogControl relop Prompt: Operator:
      mask DialogControl const Prompt: Constant value:
      mask DialogControl OutDataTypeStr Prompt: Output data type:
      mask DialogControl ZeroCross Prompt: Enable zero-crossing detection
      mask Display: disp(str)
  Constant{1..8} (8 alike) : Constant  OutDataTypeStr=boolean
  Covariance Matrix : Subsystem
      settings: PortSchema="{\"entries\":[{\"content\":{\"sides\":[{\"content\":{\"connectorIds\":[\"In1\",\"In2\",\"In3\",\"In4\",\"In5\",\"In6\",\"In7\",\"In8\"]},\"type\":\"ConnectorPlacement.EquallySpacedRectSide\",\"uuid\":\"8604b8bd-6437-4f61-845f-68e8b5fac389\"},{\"content\":{\"connectorIds\":[\"Out1\",\"Out2\",\"Out3\",\"Out4\",\"Out5\",\"Out6\"],\"side\":\"RIGHT\"},\"type\":\"ConnectorPlacement.EquallySpacedRectSide\",\"uuid\":\"d39fd40c-d67e-46d5-b0a8-3014e1ecc186\"},{\"content\":{\"connectorIds\":[\"In9\"],\"side\":\"TOP\"},\"type\":\"ConnectorPlacement.EquallySpacedRectSide\",\"uuid\":\"4f74e432-20d9-4ae9-a889-27e37d930d6f\"},{\"content\":{\"side\":\"BOTTOM\"},\"type\":\"ConnectorPlacement.EquallySpacedRectSide\",\"uuid\":\"6d71da68-886d-48a5-a91d-56b84ddd4bf2\"}]},\"type\":\"ConnectorPlacement.EquallySpacedConnector\",\"uuid\":\"ca37f2c3-e85f-4529-98b4-a6b5e671d78f\"}],\"packageUris\":[\"http://schema.mathworks.com/mf0/Connector/R2020b\"],\"version\":\"1.0\"}"
  Delay{,1..5} (6 alike) : Delay  DelayLength=1  ShowEnablePort=on
      settings: InputPortMap=u0,e6
  Hardware Friendly MUSIC Algorithm : Subsystem
  I/Q Separation : Subsystem
  I/Q Separation1 : Subsystem
  I/Q Separation2 : Subsystem
  I/Q Separation3 : Subsystem
  P_theta : Outport
  Theta : Outport  Port=2
  wires:
  Covariance Matrix/2(R21_Im) -> Delay1/1
  Delay5/1 -> Hardware Friendly MUSIC Algorithm/6(R41_Im)
  Delay1/1 -> Hardware Friendly MUSIC Algorithm/2(R21_Im)
  A Constant Calculations1/3(a2_Re) -> Hardware Friendly MUSIC Algorithm/9(a2_Re)
  A Constant Calculations1/5(a3_Re) -> Hardware Friendly MUSIC Algorithm/11(a3_Re)
  Delay3/1 -> Hardware Friendly MUSIC Algorithm/4(R31_Im)
  Hardware Friendly MUSIC Algorithm/1(P_Theta) -> P_theta/1
  A Constant Calculations1/2(a1_Im) -> Hardware Friendly MUSIC Algorithm/8(a1_Im)
  Covariance Matrix/6(R41_Im) -> Delay5/1
  Delay4/1 -> Hardware Friendly MUSIC Algorithm/5(R41_Re)
  RESET/1 -> Covariance Matrix/9(RESET)
  Covariance Matrix/4(R31_Im) -> Delay3/1
  A Constant Calculations1/1(a1_Re) -> Hardware Friendly MUSIC Algorithm/7(a1_Re)
  Compare To Constant/1(y) -> Delay5/2, Delay/2, Delay1/2, Delay2/2, Delay3/2, Delay4/2
  Covariance Matrix/5(R41_Re) -> Delay4/1
  Delay/1 -> Hardware Friendly MUSIC Algorithm/1(R21_Re)
  A Constant Calculations1/4(a2_Im) -> Hardware Friendly MUSIC Algorithm/10(a2_Im)
  Delay2/1 -> Hardware Friendly MUSIC Algorithm/3(R31_Re)
  Covariance Matrix/1(R21_Re) -> Delay/1
  A Constant Calculations1/7(Index) -> Compare To Constant/1(u), Theta/1
  Covariance Matrix/3(R31_Re) -> Delay2/1
  A Constant Calculations1/6(a3_Im) -> Hardware Friendly MUSIC Algorithm/12(a3_Im)
  F0 Index/1 -> I/Q Separation1/2(F0 Index), I/Q Separation3/2(F0 Index), A Constant Calculations1/1(F0 Index), I/Q Separation2/2(F0 Index), I/Q Separation/2(F0 Index)
  IQ Counter/1 -> I/Q Separation3/3(IQ Counter Input), I/Q Separation2/3(IQ Counter Input), I/Q Separation1/3(IQ Counter Input), I/Q Separation/3(IQ Counter Input)
  Mic1/1 -> I/Q Separation/1(Microphone Input)
  Mic2/1 -> I/Q Separation1/1(Microphone Input)
  Mic3/1 -> I/Q Separation2/1(Microphone Input)
  Mic4/1 -> I/Q Separation3/1(Microphone Input)
  A Counter/1 -> A Constant Calculations1/2(A Counter)
  I/Q Separation/1(I[n]) -> Biquad Filter1/1(dataIn)
  Constant1/1 -> Biquad Filter1/2(validIn)
  Biquad Filter1/1(dataOut) -> Covariance Matrix/1(X1_Re)
  I/Q Separation1/1(I[n]) -> Biquad Filter2/1(dataIn)
  Constant2/1 -> Biquad Filter2/2(validIn)
  Biquad Filter2/1(dataOut) -> Covariance Matrix/3(X2_Re)
  I/Q Separation1/2(Q[n]) -> Biquad Filter3/1(dataIn)
  Constant3/1 -> Biquad Filter3/2(validIn)
  Biquad Filter3/1(dataOut) -> Covariance Matrix/4(X2_Im)
  I/Q Separation/2(Q[n]) -> Biquad Filter4/1(dataIn)
  Constant8/1 -> Biquad Filter4/2(validIn)
  Biquad Filter4/1(dataOut) -> Covariance Matrix/2(X1_Im)
  I/Q Separation2/1(I[n]) -> Biquad Filter5/1(dataIn)
  Constant4/1 -> Biquad Filter5/2(validIn)
  Biquad Filter5/1(dataOut) -> Covariance Matrix/5(X3_Re)
  I/Q Separation2/2(Q[n]) -> Biquad Filter6/1(dataIn)
  Constant5/1 -> Biquad Filter6/2(validIn)
  Biquad Filter6/1(dataOut) -> Covariance Matrix/6(X3_Im)
  I/Q Separation3/1(I[n]) -> Biquad Filter7/1(dataIn)
  Constant6/1 -> Biquad Filter7/2(validIn)
  Biquad Filter7/1(dataOut) -> Covariance Matrix/7(X4_Re)
  I/Q Separation3/2(Q[n]) -> Biquad Filter8/1(dataIn)
  Constant7/1 -> Biquad Filter8/2(validIn)
  Biquad Filter8/1(dataOut) -> Covariance Matrix/8(X4_Im)

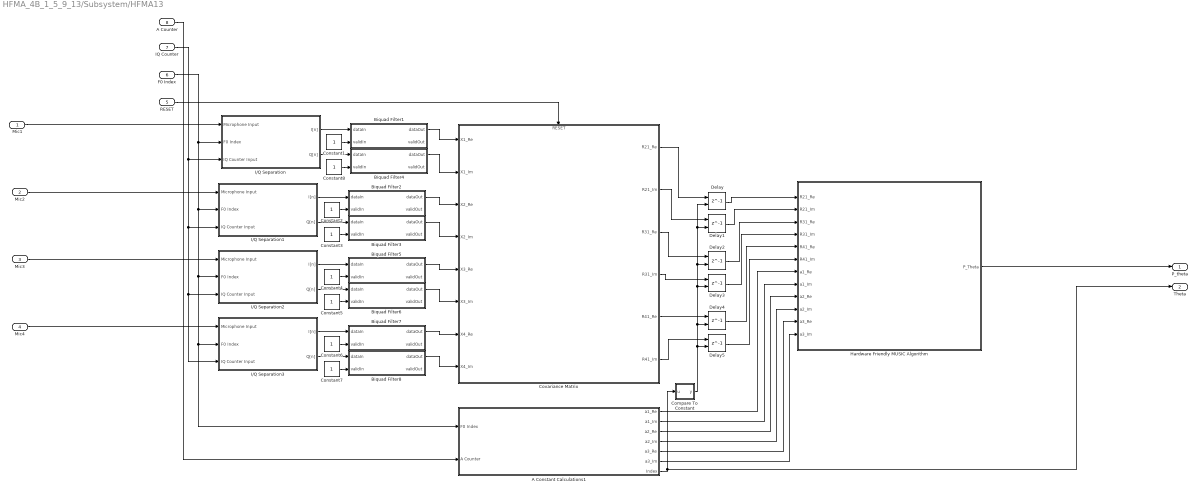
== system HFMA_4B_1_5_9_13/Subsystem/HFMA13 ==
  Mic1 : Inport
  Mic2 : Inport  Port=2
  Mic3 : Inport  Port=3
  Mic4 : Inport  Port=4
  RESET : Inport  Port=5
  F0 Index : Inport  Port=6
  IQ Counter : Inport  Port=7
  A Counter : Inport  Port=8
  A Constant Calculations1 : Subsystem
  Biquad Filter1 : Subsystem
  Biquad Filter2 : Subsystem
  Biquad Filter3 : Subsystem
  Biquad Filter4 : Subsystem
  Biquad Filter5 : Subsystem
  Biquad Filter6 : Subsystem
  Biquad Filter7 : Subsystem
  Biquad Filter8 : Subsystem
  Compare To Constant : Subsystem  mask(Compare To Constant){relop===, const=180, OutDataTypeStr=boolean, ZeroCross=on}
      mask prompts: relop "Simulink:masks:Operator_MP"; const "Simulink:masks:ConstantValue_MP"; OutDataTypeStr "Simulink:masks:OutputDataType_MP"; ZeroCross "Simulink:masks:EnableZerocrossingDetection_MP"
      mask help: Simulink:masks:CompareToConstant_MD
      mask init: same as HFMA_4B_1_5_9_13/Subsystem/HFMA1/Compare To Constant
      mask TypeOptions relop: == | ~= | < | <= | >= | >
      mask TypeOptions OutDataTypeStr: Simulink:masks:uint8 | Simulink:masks:boolean
      mask Callback ZeroCross: sl('zeroCrossEnable', gcbh);
      mask DialogControl relop Prompt: Operator:
      mask DialogControl const Prompt: Constant value:
      mask DialogControl OutDataTypeStr Prompt: Output data type:
      mask DialogControl ZeroCross Prompt: Enable zero-crossing detection
      mask Display: disp(str)
  Constant{1..8} (8 alike) : Constant  OutDataTypeStr=boolean
  Covariance Matrix : Subsystem
      settings: PortSchema="{\"entries\":[{\"content\":{\"sides\":[{\"content\":{\"connectorIds\":[\"In1\",\"In2\",\"In3\",\"In4\",\"In5\",\"In6\",\"In7\",\"In8\"]},\"type\":\"ConnectorPlacement.EquallySpacedRectSide\",\"uuid\":\"8604b8bd-6437-4f61-845f-68e8b5fac389\"},{\"content\":{\"connectorIds\":[\"Out1\",\"Out2\",\"Out3\",\"Out4\",\"Out5\",\"Out6\"],\"side\":\"RIGHT\"},\"type\":\"ConnectorPlacement.EquallySpacedRectSide\",\"uuid\":\"d39fd40c-d67e-46d5-b0a8-3014e1ecc186\"},{\"content\":{\"connectorIds\":[\"In9\"],\"side\":\"TOP\"},\"type\":\"ConnectorPlacement.EquallySpacedRectSide\",\"uuid\":\"4f74e432-20d9-4ae9-a889-27e37d930d6f\"},{\"content\":{\"side\":\"BOTTOM\"},\"type\":\"ConnectorPlacement.EquallySpacedRectSide\",\"uuid\":\"6d71da68-886d-48a5-a91d-56b84ddd4bf2\"}]},\"type\":\"ConnectorPlacement.EquallySpacedConnector\",\"uuid\":\"ca37f2c3-e85f-4529-98b4-a6b5e671d78f\"}],\"packageUris\":[\"http://schema.mathworks.com/mf0/Connector/R2020b\"],\"version\":\"1.0\"}"
  Delay{,1..5} (6 alike) : Delay  DelayLength=1  ShowEnablePort=on
      settings: InputPortMap=u0,e6
  Hardware Friendly MUSIC Algorithm : Subsystem
  I/Q Separation : Subsystem
  I/Q Separation1 : Subsystem
  I/Q Separation2 : Subsystem
  I/Q Separation3 : Subsystem
  P_theta : Outport
  Theta : Outport  Port=2
  wires:
  Covariance Matrix/2(R21_Im) -> Delay1/1
  Delay5/1 -> Hardware Friendly MUSIC Algorithm/6(R41_Im)
  Delay1/1 -> Hardware Friendly MUSIC Algorithm/2(R21_Im)
  A Constant Calculations1/3(a2_Re) -> Hardware Friendly MUSIC Algorithm/9(a2_Re)
  A Constant Calculations1/5(a3_Re) -> Hardware Friendly MUSIC Algorithm/11(a3_Re)
  Delay3/1 -> Hardware Friendly MUSIC Algorithm/4(R31_Im)
  Hardware Friendly MUSIC Algorithm/1(P_Theta) -> P_theta/1
  A Constant Calculations1/2(a1_Im) -> Hardware Friendly MUSIC Algorithm/8(a1_Im)
  Covariance Matrix/6(R41_Im) -> Delay5/1
  Delay4/1 -> Hardware Friendly MUSIC Algorithm/5(R41_Re)
  RESET/1 -> Covariance Matrix/9(RESET)
  Covariance Matrix/4(R31_Im) -> Delay3/1
  A Constant Calculations1/1(a1_Re) -> Hardware Friendly MUSIC Algorithm/7(a1_Re)
  Compare To Constant/1(y) -> Delay5/2, Delay/2, Delay1/2, Delay2/2, Delay3/2, Delay4/2
  Covariance Matrix/5(R41_Re) -> Delay4/1
  Delay/1 -> Hardware Friendly MUSIC Algorithm/1(R21_Re)
  A Constant Calculations1/4(a2_Im) -> Hardware Friendly MUSIC Algorithm/10(a2_Im)
  Delay2/1 -> Hardware Friendly MUSIC Algorithm/3(R31_Re)
  Covariance Matrix/1(R21_Re) -> Delay/1
  A Constant Calculations1/7(Index) -> Compare To Constant/1(u), Theta/1
  Covariance Matrix/3(R31_Re) -> Delay2/1
  A Constant Calculations1/6(a3_Im) -> Hardware Friendly MUSIC Algorithm/12(a3_Im)
  F0 Index/1 -> I/Q Separation1/2(F0 Index), I/Q Separation3/2(F0 Index), A Constant Calculations1/1(F0 Index), I/Q Separation2/2(F0 Index), I/Q Separation/2(F0 Index)
  IQ Counter/1 -> I/Q Separation3/3(IQ Counter Input), I/Q Separation2/3(IQ Counter Input), I/Q Separation1/3(IQ Counter Input), I/Q Separation/3(IQ Counter Input)
  Mic1/1 -> I/Q Separation/1(Microphone Input)
  Mic2/1 -> I/Q Separation1/1(Microphone Input)
  Mic3/1 -> I/Q Separation2/1(Microphone Input)
  Mic4/1 -> I/Q Separation3/1(Microphone Input)
  A Counter/1 -> A Constant Calculations1/2(A Counter)
  I/Q Separation/1(I[n]) -> Biquad Filter1/1(dataIn)
  Constant1/1 -> Biquad Filter1/2(validIn)
  Biquad Filter1/1(dataOut) -> Covariance Matrix/1(X1_Re)
  I/Q Separation1/1(I[n]) -> Biquad Filter2/1(dataIn)
  Constant2/1 -> Biquad Filter2/2(validIn)
  Biquad Filter2/1(dataOut) -> Covariance Matrix/3(X2_Re)
  I/Q Separation1/2(Q[n]) -> Biquad Filter3/1(dataIn)
  Constant3/1 -> Biquad Filter3/2(validIn)
  Biquad Filter3/1(dataOut) -> Covariance Matrix/4(X2_Im)
  I/Q Separation/2(Q[n]) -> Biquad Filter4/1(dataIn)
  Constant8/1 -> Biquad Filter4/2(validIn)
  Biquad Filter4/1(dataOut) -> Covariance Matrix/2(X1_Im)
  I/Q Separation2/1(I[n]) -> Biquad Filter5/1(dataIn)
  Constant4/1 -> Biquad Filter5/2(validIn)
  Biquad Filter5/1(dataOut) -> Covariance Matrix/5(X3_Re)
  I/Q Separation2/2(Q[n]) -> Biquad Filter6/1(dataIn)
  Constant5/1 -> Biquad Filter6/2(validIn)
  Biquad Filter6/1(dataOut) -> Covariance Matrix/6(X3_Im)
  I/Q Separation3/1(I[n]) -> Biquad Filter7/1(dataIn)
  Constant6/1 -> Biquad Filter7/2(validIn)
  Biquad Filter7/1(dataOut) -> Covariance Matrix/7(X4_Re)
  I/Q Separation3/2(Q[n]) -> Biquad Filter8/1(dataIn)
  Constant7/1 -> Biquad Filter8/2(validIn)
  Biquad Filter8/1(dataOut) -> Covariance Matrix/8(X4_Im)

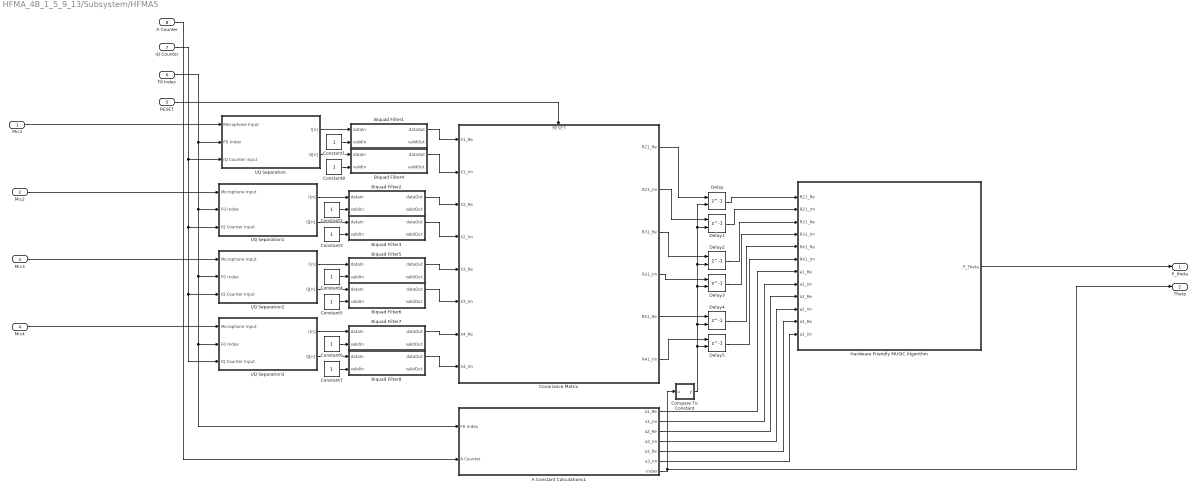
== system HFMA_4B_1_5_9_13/Subsystem/HFMA5 ==
  Mic1 : Inport
  Mic2 : Inport  Port=2
  Mic3 : Inport  Port=3
  Mic4 : Inport  Port=4
  RESET : Inport  Port=5
  F0 Index : Inport  Port=6
  IQ Counter : Inport  Port=7
  A Counter : Inport  Port=8
  A Constant Calculations1 : Subsystem
  Biquad Filter1 : Subsystem
  Biquad Filter2 : Subsystem
  Biquad Filter3 : Subsystem
  Biquad Filter4 : Subsystem
  Biquad Filter5 : Subsystem
  Biquad Filter6 : Subsystem
  Biquad Filter7 : Subsystem
  Biquad Filter8 : Subsystem
  Compare To Constant : Subsystem  mask(Compare To Constant){relop===, const=180, OutDataTypeStr=boolean, ZeroCross=on}
      mask prompts: relop "Simulink:masks:Operator_MP"; const "Simulink:masks:ConstantValue_MP"; OutDataTypeStr "Simulink:masks:OutputDataType_MP"; ZeroCross "Simulink:masks:EnableZerocrossingDetection_MP"
      mask help: Simulink:masks:CompareToConstant_MD
      mask init: same as HFMA_4B_1_5_9_13/Subsystem/HFMA1/Compare To Constant
      mask TypeOptions relop: == | ~= | < | <= | >= | >
      mask TypeOptions OutDataTypeStr: Simulink:masks:uint8 | Simulink:masks:boolean
      mask Callback ZeroCross: sl('zeroCrossEnable', gcbh);
      mask DialogControl relop Prompt: Operator:
      mask DialogControl const Prompt: Constant value:
      mask DialogControl OutDataTypeStr Prompt: Output data type:
      mask DialogControl ZeroCross Prompt: Enable zero-crossing detection
      mask Display: disp(str)
  Constant{1..8} (8 alike) : Constant  OutDataTypeStr=boolean
  Covariance Matrix : Subsystem
      settings: PortSchema="{\"entries\":[{\"content\":{\"sides\":[{\"content\":{\"connectorIds\":[\"In1\",\"In2\",\"In3\",\"In4\",\"In5\",\"In6\",\"In7\",\"In8\"]},\"type\":\"ConnectorPlacement.EquallySpacedRectSide\",\"uuid\":\"8604b8bd-6437-4f61-845f-68e8b5fac389\"},{\"content\":{\"connectorIds\":[\"Out1\",\"Out2\",\"Out3\",\"Out4\",\"Out5\",\"Out6\"],\"side\":\"RIGHT\"},\"type\":\"ConnectorPlacement.EquallySpacedRectSide\",\"uuid\":\"d39fd40c-d67e-46d5-b0a8-3014e1ecc186\"},{\"content\":{\"connectorIds\":[\"In9\"],\"side\":\"TOP\"},\"type\":\"ConnectorPlacement.EquallySpacedRectSide\",\"uuid\":\"4f74e432-20d9-4ae9-a889-27e37d930d6f\"},{\"content\":{\"side\":\"BOTTOM\"},\"type\":\"ConnectorPlacement.EquallySpacedRectSide\",\"uuid\":\"6d71da68-886d-48a5-a91d-56b84ddd4bf2\"}]},\"type\":\"ConnectorPlacement.EquallySpacedConnector\",\"uuid\":\"ca37f2c3-e85f-4529-98b4-a6b5e671d78f\"}],\"packageUris\":[\"http://schema.mathworks.com/mf0/Connector/R2020b\"],\"version\":\"1.0\"}"
  Delay{,1..5} (6 alike) : Delay  DelayLength=1  ShowEnablePort=on
      settings: InputPortMap=u0,e6
  Hardware Friendly MUSIC Algorithm : Subsystem
  I/Q Separation : Subsystem
  I/Q Separation1 : Subsystem
  I/Q Separation2 : Subsystem
  I/Q Separation3 : Subsystem
  P_theta : Outport
  Theta : Outport  Port=2
  wires:
  Covariance Matrix/2(R21_Im) -> Delay1/1
  Delay5/1 -> Hardware Friendly MUSIC Algorithm/6(R41_Im)
  Delay1/1 -> Hardware Friendly MUSIC Algorithm/2(R21_Im)
  A Constant Calculations1/3(a2_Re) -> Hardware Friendly MUSIC Algorithm/9(a2_Re)
  A Constant Calculations1/5(a3_Re) -> Hardware Friendly MUSIC Algorithm/11(a3_Re)
  Delay3/1 -> Hardware Friendly MUSIC Algorithm/4(R31_Im)
  Hardware Friendly MUSIC Algorithm/1(P_Theta) -> P_theta/1
  A Constant Calculations1/2(a1_Im) -> Hardware Friendly MUSIC Algorithm/8(a1_Im)
  Covariance Matrix/6(R41_Im) -> Delay5/1
  Delay4/1 -> Hardware Friendly MUSIC Algorithm/5(R41_Re)
  RESET/1 -> Covariance Matrix/9(RESET)
  Covariance Matrix/4(R31_Im) -> Delay3/1
  A Constant Calculations1/1(a1_Re) -> Hardware Friendly MUSIC Algorithm/7(a1_Re)
  Compare To Constant/1(y) -> Delay5/2, Delay/2, Delay1/2, Delay2/2, Delay3/2, Delay4/2
  Covariance Matrix/5(R41_Re) -> Delay4/1
  Delay/1 -> Hardware Friendly MUSIC Algorithm/1(R21_Re)
  A Constant Calculations1/4(a2_Im) -> Hardware Friendly MUSIC Algorithm/10(a2_Im)
  Delay2/1 -> Hardware Friendly MUSIC Algorithm/3(R31_Re)
  Covariance Matrix/1(R21_Re) -> Delay/1
  A Constant Calculations1/7(Index) -> Compare To Constant/1(u), Theta/1
  Covariance Matrix/3(R31_Re) -> Delay2/1
  A Constant Calculations1/6(a3_Im) -> Hardware Friendly MUSIC Algorithm/12(a3_Im)
  F0 Index/1 -> I/Q Separation1/2(F0 Index), I/Q Separation3/2(F0 Index), A Constant Calculations1/1(F0 Index), I/Q Separation2/2(F0 Index), I/Q Separation/2(F0 Index)
  IQ Counter/1 -> I/Q Separation3/3(IQ Counter Input), I/Q Separation2/3(IQ Counter Input), I/Q Separation1/3(IQ Counter Input), I/Q Separation/3(IQ Counter Input)
  Mic1/1 -> I/Q Separation/1(Microphone Input)
  Mic2/1 -> I/Q Separation1/1(Microphone Input)
  Mic3/1 -> I/Q Separation2/1(Microphone Input)
  Mic4/1 -> I/Q Separation3/1(Microphone Input)
  A Counter/1 -> A Constant Calculations1/2(A Counter)
  I/Q Separation/1(I[n]) -> Biquad Filter1/1(dataIn)
  Constant1/1 -> Biquad Filter1/2(validIn)
  Biquad Filter1/1(dataOut) -> Covariance Matrix/1(X1_Re)
  I/Q Separation1/1(I[n]) -> Biquad Filter2/1(dataIn)
  Constant2/1 -> Biquad Filter2/2(validIn)
  Biquad Filter2/1(dataOut) -> Covariance Matrix/3(X2_Re)
  I/Q Separation1/2(Q[n]) -> Biquad Filter3/1(dataIn)
  Constant3/1 -> Biquad Filter3/2(validIn)
  Biquad Filter3/1(dataOut) -> Covariance Matrix/4(X2_Im)
  I/Q Separation/2(Q[n]) -> Biquad Filter4/1(dataIn)
  Constant8/1 -> Biquad Filter4/2(validIn)
  Biquad Filter4/1(dataOut) -> Covariance Matrix/2(X1_Im)
  I/Q Separation2/1(I[n]) -> Biquad Filter5/1(dataIn)
  Constant4/1 -> Biquad Filter5/2(validIn)
  Biquad Filter5/1(dataOut) -> Covariance Matrix/5(X3_Re)
  I/Q Separation2/2(Q[n]) -> Biquad Filter6/1(dataIn)
  Constant5/1 -> Biquad Filter6/2(validIn)
  Biquad Filter6/1(dataOut) -> Covariance Matrix/6(X3_Im)
  I/Q Separation3/1(I[n]) -> Biquad Filter7/1(dataIn)
  Constant6/1 -> Biquad Filter7/2(validIn)
  Biquad Filter7/1(dataOut) -> Covariance Matrix/7(X4_Re)
  I/Q Separation3/2(Q[n]) -> Biquad Filter8/1(dataIn)
  Constant7/1 -> Biquad Filter8/2(validIn)
  Biquad Filter8/1(dataOut) -> Covariance Matrix/8(X4_Im)
